simulink model "ElectroMechanics_Q"  (R2024b)
settings: Solver=VariableStepAuto  StartTime=0.0  StopTime=10.0  RelTol=1e-3
libraries: fl_lib x5, nesl_utility x5, sdl_lib x1, batteryecm_lib x1, ee_lib x1
settings Model: Creator=hp  LastModifiedBy=hp

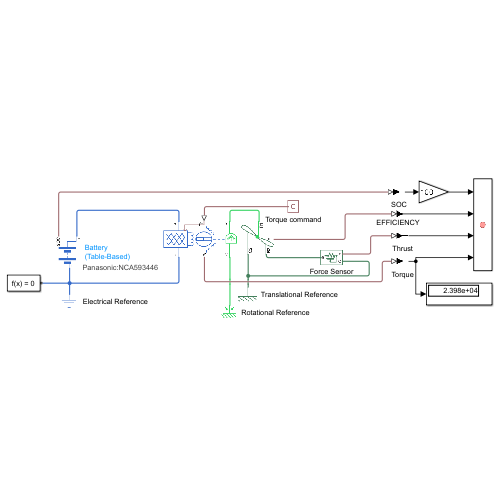
[thumbnail: Simulink's stored preview of the top-level diagram]
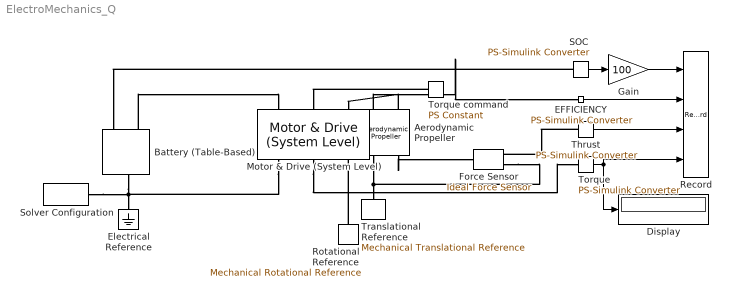
== system ElectroMechanics_Q ==
  " Electrical Reference" : fl_lib/Electrical/Electrical Elements/Electrical Reference
  Aerodynamic Propeller : sdl_lib/Engines & Motors/Aerodynamic Propeller  parameterization=sdl.enum.AerodynamicPropellerParameterization.Constant  pitch_type=foundation.enum.constant_controlled.constant  direction=sdl.enum.PropellerDirection.Positive  root_pitch=0 deg  D=.057 m  kt_const=.1  kp_const=.05  kt_poly_fixed=[.002, .0006, -.0509, .0617]  kp_poly_fixed=[-.0752, .0577, -.0622, .16]  pitch_angle_TLU=[-15, 15, 25, 35, 45] deg  kt_poly_TLU=[.0002, -.00041, -.036, .03; .00026, -.00056, -.048, .04; .002, .00063, -.051, .062; .0014, -.0016, -.048, .087; .00087, -.0036, -.041, .12]  kp_poly_TLU=[-.1, .031, .0055, .088; -.081, -.025, .0044, .07; -.075, .058, -.062, .16; -.052, .065, -.08, .3; -.031, .057, -.069, .4]  J_TLU=[.01, .3, .625, 1.55, 2, 2.6]  kt_TLU_1D=[.0614, .0473, .0318, -.0127, -.0343, -.063]  kp_TLU_1D=[.1496, .1314, .116, -.0521, -.1503, -.2813]  kt_TLU_2D=[.00019, .013, .0048, -.017, -.03, -.045; .00039, .025, .0096, -.037, -.06, -.09; .00061, .047, .032, -.013, -.034, -.063; .00086, .072, .057, .014, -.0076, -.036; .12, .104, .09, .049, .029, .0019]  kp_TLU_2D=[.029, .029, .016, .06, .009, -.16; .059, .054, .031, -.12, -.19, -.29; .15, .13, .12, -.052, -.15, -.28; .26, .24, .22, .097, -.04, -.25; .39, .39, .38, .32, .24, .062]  beta_TLU=linspace(0, 360, 10) deg  Ct_TLU_1D=0.035 * sind(linspace(0, 360, 10) - 200)  Cq_TLU_1D=0.010 * sind(linspace(0, 360, 10) - 200)  Ct_TLU_2D=[0.01 * sind(linspace(0, 360, 10) - 200); 0.020 * sind(linspace(0, 360, 10) - 200); 0.035 * sind(linspace(0, 360, 10) - 200); 0.04 * sind(linspace(0, 360, 10) - 200); 0.06 * sind(linspace(0, 360, 10) - 200)]  Cq_TLU_2D=[0.0005 * sind(linspace(0, 360, 10) - 200); 0.0015 * sind(linspace(0, 360, 10) - 200); 0.0025 * sind(linspace(0, 360, 10) - 200); 0.0035 * sind(linspace(0, 360, 10) - 200); 0.0045 * sind(linspace(0, 360, 10) - 200)]  n_blades=2  n_blade_discretization=20  radial_TLU=[.1, .12, .2, .4, .6, .8, 1]  twist_TLU=[30, 35, 50, 30, 20, 15, 10] deg  chord_TLU=[.0676, .0666, .0824, .1025, .0885, .0598, .0133]  alpha_TLU=-180 : 10 : 180 deg  Cl_TLU=[.1326, .1326, .1274, .1274, .1274, .1274, .1274; .3626, .3626, .5002, .5002, .5002, .5002, .5002; .5528, .5528, .8007, .8007, .8007, .8007, .8007; .7256, .7256, 1.0125, 1.0125, 1.0125, 1.0125, 1.0125; .8016, .8016, 1.1556, 1.1556, 1.1556, 1.1556, 1.1556; .7873, .7873, 1.1604, 1.1604, 1.1604, 1.1604, 1.1604; .7031, .7031, 1.0493, 1.0493, 1.0493, 1.0493, 1.0493; .5423, .5423, .7973, .7973, .7973, .7973, .7973; .3537, .3537, .4332, .4332, .4332, .4332, .4332; .1155, .1155, -.0376, -.0376, -.0376, -.0376, -.0376; -.1045, -.1045, -.4096, -.4096, -.4096, -.4096, -.4096; -.2999, -.2999, -.672, -.672, -.672, -.672, -.672; -.4401, -.4401, -.9343, -.9343, -.9343, -.9343, -.9343; -.5186, -.5186, -1.0477, -1.0477, -1.0477, -1.0477, -1.0477; -.5303, -.5303, -1.0387, -1.0387, -1.0387, -1.0387, -1.0387; -.5073, -.5073, -.9565, -.9565, -.9565, -.9565, -.9565; -.442, -.442, -.7713, -.7713, -.7713, -.7713, -.7713; -.2658, -.2658, -.4832, -.4832, -.4832, -.4832, -.4832; .4109, .4109, .3629, .3629, .3629, .3629, .3629; 1.1635, 1.1635, 1.3779, 1.3779, 1.3779, 1.3779, 1.3779; 1.2412, 1.2412, 1.4033, 1.4033, 1.4033, 1.4033, 1.4033; .7434, .7434, 1.3453, 1.3453, 1.3453, 1.3453, 1.3453; .7908, .7908, 1.2862, 1.2862, 1.2862, 1.2862, 1.2862; .7525, .7525, 1.1562, 1.1562, 1.1562, 1.1562, 1.1562; .6722, .6722, .9487, .9487, .9487, .9487, .9487; .5324, .5324, .7047, .7047, .7047, .7047, .7047; .3365, .3365, .382, .382, .382, .382, .382; .0529, .0529, -.0229, -.0229, -.0229, -.0229, -.0229; -.2728, -.2728, -.316, -.316, -.316, -.316, -.316; -.4135, -.4135, -.6195, -.6195, -.6195, -.6195, -.6195; -.5087, -.5087, -.7847, -.7847, -.7847, -.7847, -.7847; -.5342, -.5342, -.8419, -.8419, -.8419, -.8419, -.8419; -.5166, -.5166, -.7658, -.7658, -.7658, -.7658, -.7658; -.4321, -.4321, -.5707, -.5707, -.5707, -.5707, -.5707; -.2864, -.2864, -.3098, -.3098, -.3098, -.3098, -.3098; -.1073, -.1073, -.0893, -.0893, -.0893, -.0893, -.0893; .1326, .1326, .1274, .1274, .1274, .1274, .1274]  Cd_TLU=[.0055, .0055, .3904, .3904, .3904, .3904, .3904; .0774, .0774, .449, .449, .449, .449, .449; .2412, .2412, .5915, .5915, .5915, .5915, .5915; .4342, .4342, .8307, .8307, .8307, .8307, .8307; .679, .679, 1.0909, 1.0909, 1.0909, 1.0909, 1.0909; .9003, .9003, 1.3868, 1.3868, 1.3868, 1.3868, 1.3868; 1.0825, 1.0825, 1.6565, 1.6565, 1.6565, 1.6565, 1.6565; 1.2281, 1.2281, 1.875, 1.875, 1.875, 1.875, 1.875; 1.3205, 1.3205, 2.017, 2.017, 2.017, 2.017, 2.017; 1.3234, 1.3234, 2.0407, 2.0407, 2.0407, 2.0407, 2.0407; 1.2391, 1.2391, 1.9513, 1.9513, 1.9513, 1.9513, 1.9513; 1.0963, 1.0963, 1.7643, 1.7643, 1.7643, 1.7643, 1.7643; .8978, .8978, 1.5048, 1.5048, 1.5048, 1.5048, 1.5048; .6525, .6525, 1.2281, 1.2281, 1.2281, 1.2281, 1.2281; .4203, .4203, .838, .838, .838, .838, .838; .2428, .2428, .5434, .5434, .5434, .5434, .5434; .0951, .0951, .2517, .2517, .2517, .2517, .2517; .0292, .0292, .0698, .0698, .0698, .0698, .0698; .0148, .0148, .0267, .0267, .0267, .0267, .0267; .0808, .0808, .0509, .0509, .0509, .0509, .0509; .2429, .2429, .1561, .1561, .1561, .1561, .1561; .5019, .5019, .3927, .3927, .3927, .3927, .3927; .7217, .7217, .7438, .7438, .7438, .7438, .7438; .9336, .9336, 1.1277, 1.1277, 1.1277, 1.1277, 1.1277; 1.0984, 1.0984, 1.4838, 1.4838, 1.4838, 1.4838, 1.4838; 1.2274, 1.2274, 1.7877, 1.7877, 1.7877, 1.7877, 1.7877; 1.3016, 1.3016, 1.9779, 1.9779, 1.9779, 1.9779, 1.9779; 1.3305, 1.3305, 2.0516, 2.0516, 2.0516, 2.0516, 2.0516; 1.2889, 1.2889, 1.9974, 1.9974, 1.9974, 1.9974, 1.9974; 1.1677, 1.1677, 1.8463, 1.8463, 1.8463, 1.8463, 1.8463; 1.0076, 1.0076, 1.5699, 1.5699, 1.5699, 1.5699, 1.5699; .8068, .8068, 1.2596, 1.2596, 1.2596, 1.2596, 1.2596; .5688, .5688, .9493, .9493, .9493, .9493, .9493; .3604, .3604, .6154, .6154, .6154, .6154, .6154; .1802, .1802, .5015, .5015, .5015, .5015, .5015; .0699, .0699, .4265, .4265, .4265, .4265, .4265; .0055, .0055, .3904, .3904, .3904, .3904, .3904]  interp_method=simscape.enum.interpolation.linear  extrap_method=simscape.enum.extrapolation.linear  density_spec=foundation.enum.constant_variable.constant  rho=1.225 kg/m^3  rotational_ports=sdl.enum.ConnectionType.Conserving  translational_ports=sdl.enum.ConnectionType.Conserving  model_inertia=true  propeller_inertia=1.5e-7 kg*m^2  propeller_mass=.5 g  efficiency_sensor=true  n_thr=0.001 Hz  k_thr=0.001  P_thr=0.01 W  operation_check=simscape.enum.assert.action.warn  expose_port_C=false  w_specify=off  w_priority=None  w=0 rad/s  w_nominal_specify=off  w_nominal_value=1  w_nominal_unit=rad/s  Q_specify=off  Q_priority=None  Q=0 N*m  Q_nominal_specify=off  Q_nominal_value=1  Q_nominal_unit=N*m  v_specify=off  v_priority=None  v=0 m/s  v_nominal_specify=off  v_nominal_value=1  v_nominal_unit=m/s  thrust_specify=off  thrust_priority=None  thrust=0 N  thrust_nominal_specify=on  thrust_nominal_value=1  thrust_nominal_unit=N
      settings: InternalSimscapePortConfiguration="{\"Bottom\":[],\"Left\":[{\"id\":\"R1\",\"label\":\"R1\",\"type\":\"foundation.mechanical.rotational.rotational\"}],\"Right\":[{\"id\":\"R2\",\"label\":\"R2\",\"type\":\"foundation.mechanical.translational.translational\"},{\"id\":\"C2\",\"label\":\"C2\",\"type\":\"foundation.mechanical.translational.translational\"}],\"Top\":[{\"id\":\"Eff_out\",\"label\":\"E\",\"type\":\"output\"}]}"
  Battery (Table-Based) : batteryecm_lib/Battery (Table-Based)  PartSpecification="{\"DatasetId\":\"Panasonic|NCA593446|simscape.battery.batteryTableBased\",\"DisplayName\":\"Panasonic:NCA593446\"}"  SOC_vec=[0 0.01 0.02 0.03 0.04 0.05 0.06 0.07 0.08 0.09 0.1 0.11 0.12 0.13 0.14 0.15 0.16 0.17 0.18 0.19 0.2 0.21 0.22 0.23 0.24 0.25 0.26 0.27 0.28 0.29 0.3 0.31 0.32 0.33 0.34 0.35 0.36 0.37 0.38 0.39 0.4 0.41 0.42 0.43 0.44 0.45 0.46 0.47 0.48 0.49 0.5 0.51 0.52 0.53 0.54 0.55 0.56 0.57 0.58 0.59 0.6 0.61 0.62 0.63 0.64 0.65 0.66 0.67 0.68 0.69 0.7 0.71 0.72 0.73 0.74 0.75 0.76 0.77 0.78 0.79 0.8 0.81 0.82 0.83 0.84 0.85 0.86 0.87 0.88 0.89 0.9 0.91 0.92 0.93 0.94 0.95 0.96 0.97 0.98 0.99 1] % Datasheet derived  T_dependence=simscape.enum.tablebattery.temperature_dependence.yes  prm_dir=simscape.enum.tablebattery.prm_dir.noCurrentDirectionality  T_vec=[-20 -10 0 25 40] % Datasheet derived degC  V0_mat=[2.84768 2.84768 2.84768 2.84768 2.84768;2.96826 2.96826 2.96826 2.96826 2.96826;3.06574 3.06574 3.06574 3.06574 3.06574;3.13766 3.13766 3.13766 3.13766 3.13766;3.1967 3.1967 3.1967 3.1967 3.1967;3.24166 3.24166 3.24166 3.24166 3.24166;3.27473 3.27473 3.27473 3.27473 3.27473;3.30127 3.30127 3.30127 3.30127 3.30127;3.32686 3.32686 3.32686 3.32686 3.32686;3.34997 3.34997 3.34997 3.34997 3.34997;3.37005 3.37005 3.37005 3.37005 3.37005;3.38547 3.38547 3.38547 3.38547 3.38547;3.39998 3.39998 3.39998 3.39998 3.39998;3.41477 3.41477 3.41477 3.41477 3.41477;3.42833 3.42833 3.42833 3.42833 3.42833;3.4411 3.4411 3.4411 3.4411 3.4411;3.45204 3.45204 3.45204 3.45204 3.45204;3.46216 3.46216 3.46216 3.46216 3.46216;3.47107 3.47107 3.47107 3.47107 3.47107;3.47798 3.47798 3.47798 3.47798 3.47798;3.48476 3.48476 3.48476 3.48476 3.48476;3.49146 3.49146 3.49146 3.49146 3.49146;3.49846 3.49846 3.49846 3.49846 3.49846;3.50538 3.50538 3.50538 3.50538 3.50538;3.51196 3.51196 3.51196 3.51196 3.51196;3.51856 3.51856 3.51856 3.51856 3.51856;3.52563 3.52563 3.52563 3.52563 3.52563;3.53269 3.53269 3.53269 3.53269 3.53269;3.53975 3.53975 3.53975 3.53975 3.53975;3.5468 3.5468 3.5468 3.5468 3.5468;3.55304 3.55304 3.55304 3.55304 3.55304;3.5585 3.5585 3.5585 3.5585 3.5585;3.56345 3.56345 3.56345 3.56345 3.56345;3.56808 3.56808 3.56808 3.56808 3.56808;3.57208 3.57208 3.57208 3.57208 3.57208;3.57682 3.57682 3.57682 3.57682 3.57682;3.58157 3.58157 3.58157 3.58157 3.58157;3.58747 3.58747 3.58747 3.58747 3.58747;3.59339 3.59339 3.59339 3.59339 3.59339;3.59973 3.59973 3.59973 3.59973 3.59973;3.6062 3.6062 3.6062 3.6062 3.6062;3.61263 3.61263 3.61263 3.61263 3.61263;3.61836 3.61836 3.61836 3.61836 3.61836;3.62359 3.62359 3.62359 3.62359 3.62359;3.62865 3.62865 3.62865 3.62865 3.62865;3.63358 3.63358 3.63358 3.63358 3.63358;3.63894 3.63894 3.63894 3.63894 3.63894;3.64566 3.64566 3.64566 3.64566 3.64566;3.65241 3.65241 3.65241 3.65241 3.65241;3.65921 3.65921 3.65921 3.65921 3.65921;3.66761 3.66761 3.66761 3.66761 3.66761;3.67554 3.67554 3.67554 3.67554 3.67554;3.68378 3.68378 3.68378 3.68378 3.68378;3.69229 3.69229 3.69229 3.69229 3.69229;3.70107 3.70107 3.70107 3.70107 3.70107;3.71105 3.71105 3.71105 3.71105 3.71105;3.72105 3.72105 3.72105 3.72105 3.72105;3.73022 3.73022 3.73022 3.73022 3.73022;3.73836 3.73836 3.73836 3.73836 3.73836;3.74563 3.74563 3.74563 3.74563 3.74563;3.75278 3.75278 3.75278 3.75278 3.75278;3.7608 3.7608 3.7608 3.7608 3.7608;3.77031 3.77031 3.77031 3.77031 3.77031;3.78086 3.78086 3.78086 3.78086 3.78086;3.7914 3.7914 3.7914 3.7914 3.7914;3.80194 3.80194 3.80194 3.80194 3.80194;3.81187 3.81187 3.81187 3.81187 3.81187;3.82008 3.82008 3.82008 3.82008 3.82008;3.8281 3.8281 3.8281 3.8281 3.8281;3.83612 3.83612 3.83612 3.83612 3.83612;3.84414 3.84414 3.84414 3.84414 3.84414;3.85216 3.85216 3.85216 3.85216 3.85216;3.86049 3.86049 3.86049 3.86049 3.86049;3.86887 3.86887 3.86887 3.86887 3.86887;3.87725 3.87725 3.87725 3.87725 3.87725;3.88563 3.88563 3.88563 3.88563 3.88563;3.89423 3.89423 3.89423 3.89423 3.89423;3.9041 3.9041 3.9041 3.9041 3.9041;3.91381 3.91381 3.91381 3.91381 3.91381;3.92353 3.92353 3.92353 3.92353 3.92353;3.93322 3.93322 3.93322 3.93322 3.93322;3.94362 3.94362 3.94362 3.94362 3.94362;3.95435 3.95435 3.95435 3.95435 3.95435;3.96525 3.96525 3.96525 3.96525 3.96525;3.97673 3.97673 3.97673 3.97673 3.97673;3.98856 3.98856 3.98856 3.98856 3.98856;4.00085 4.00085 4.00085 4.00085 4.00085;4.01324 4.01324 4.01324 4.01324 4.01324;4.02548 4.02548 4.02548 4.02548 4.02548;4.03638 4.03638 4.03638 4.03638 4.03638;4.04647 4.04647 4.04647 4.04647 4.04647;4.05605 4.05605 4.05605 4.05605 4.05605;4.06452 4.06452 4.06452 4.06452 4.06452;4.07272 4.07272 4.07272 4.07272 4.07272;4.08092 4.08092 4.08092 4.08092 4.08092;4.09076 4.09076 4.09076 4.09076 4.09076;4.1031 4.1031 4.1031 4.1031 4.1031;4.11565 4.11565 4.11565 4.11565 4.11565;4.12892 4.12892 4.12892 4.12892 4.12892;4.15272 4.15272 4.15272 4.15272 4.15272;4.17509 4.17509 4.17509 4.17509 4.17509] % Datasheet derived V  V0_vec=[2.84768 2.96826 3.06574 3.13766 3.1967 3.24166 3.27473 3.30127 3.32686 3.34997 3.37005 3.38547 3.39998 3.41477 3.42833 3.4411 3.45204 3.46216 3.47107 3.47798 3.48476 3.49146 3.49846 3.50538 3.51196 3.51856 3.52563 3.53269 3.53975 3.5468 3.55304 3.5585 3.56345 3.56808 3.57208 3.57682 3.58157 3.58747 3.59339 3.59973 3.6062 3.61263 3.61836 3.62359 3.62865 3.63358 3.63894 3.64566 3.65241 3.65921 3.66761 3.67554 3.68378 3.69229 3.70107 3.71105 3.72105 3.73022 3.73836 3.74563 3.75278 3.7608 3.77031 3.78086 3.7914 3.80194 3.81187 3.82008 3.8281 3.83612 3.84414 3.85216 3.86049 3.86887 3.87725 3.88563 3.89423 3.9041 3.91381 3.92353 3.93322 3.94362 3.95435 3.96525 3.97673 3.98856 4.00085 4.01324 4.02548 4.03638 4.04647 4.05605 4.06452 4.07272 4.08092 4.09076 4.1031 4.11565 4.12892 4.15272 4.17509] % Datasheet derived V  V_range=[2.475 Inf] % Datasheet derived V  R0_mat=[1.17152 1.25921 0.69508 0.13304 0.07171;1.17152 1.25921 1.0047 0.16124 0.03357;1.17152 1.25921 0.97374 0.17824 0.03753;1.17152 1.25921 0.94277 0.18397 0.03713;1.17152 1.25921 0.91181 0.1856 0.05177;1.17152 1.25921 0.88084 0.18421 0.05939;1.17152 1.25921 0.84988 0.17878 0.06959;1.17152 1.25921 0.81891 0.17634 0.07461;1.17152 1.25921 0.78795 0.174 0.0797;1.17152 1.25921 0.75698 0.17214 0.08635;1.17152 1.25921 0.72602 0.17223 0.0906;1.17152 1.25921 0.69505 0.17054 0.09115;1.17152 1.25921 0.66409 0.16925 0.09318;1.17152 1.22525 0.63312 0.16875 0.09628;1.17152 1.19128 0.60216 0.16787 0.0984;1.17152 1.15732 0.57119 0.16678 0.09989;1.17152 1.12335 0.54023 0.16513 0.10147;1.17152 1.08939 0.50867 0.16406 0.10281;1.17152 1.05543 0.47797 0.1625 0.10317;1.17152 1.02146 0.45459 0.15994 0.10196;1.17152 0.9875 0.43292 0.15714 0.10068;1.17152 0.95353 0.41305 0.15431 0.1;1.17152 0.91957 0.39342 0.15202 0.09955;1.17152 0.8856 0.37945 0.15067 0.09904;1.17152 0.85164 0.36632 0.14936 0.09823;1.17152 0.81767 0.35357 0.14805 0.09731;1.17152 0.78371 0.34176 0.14694 0.09677;1.17152 0.74975 0.33164 0.14582 0.09621;1.17152 0.71578 0.32415 0.14471 0.09565;1.17152 0.68182 0.31666 0.1436 0.0951;1.17152 0.64785 0.30853 0.14232 0.09389;1.17152 0.61389 0.3006 0.1409 0.09207;1.17152 0.58003 0.29425 0.13954 0.08984;1.17152 0.55268 0.28763 0.13803 0.08736;1.17152 0.52745 0.28052 0.13616 0.08533;1.17152 0.50643 0.27473 0.13458 0.08451;1.17152 0.48959 0.26905 0.133 0.08369;1.17152 0.47408 0.26428 0.1317 0.0838;1.13618 0.45924 0.26068 0.13039 0.08392;1.10083 0.44473 0.25775 0.12929 0.08436;1.06549 0.43413 0.25494 0.12827 0.0845;1.03015 0.42448 0.25209 0.12722 0.08303;0.99481 0.41337 0.2484 0.12629 0.081;0.95946 0.39916 0.24286 0.12491 0.07858;0.92412 0.38482 0.23717 0.12342 0.07601;0.88878 0.37516 0.23139 0.12187 0.07336;0.85344 0.36733 0.22594 0.12033 0.07168;0.8181 0.3606 0.22242 0.11873 0.07131;0.78275 0.35376 0.21949 0.11718 0.07096;0.74741 0.34688 0.21659 0.11566 0.07065;0.71207 0.34128 0.21496 0.11527 0.07161;0.67646 0.3359 0.21296 0.11494 0.07097;0.6411 0.33115 0.21127 0.11474 0.07051;0.61079 0.32663 0.21087 0.11476 0.07027;0.59072 0.32333 0.21068 0.11496 0.07026;0.5716 0.32098 0.21144 0.11526 0.07193;0.5582 0.31868 0.21222 0.11533 0.07363;0.54553 0.31584 0.20998 0.11502 0.07466;0.53204 0.31219 0.20683 0.11406 0.07488;0.52092 0.30767 0.20299 0.11322 0.07396;0.51011 0.30183 0.19905 0.11239 0.0719;0.49999 0.29668 0.19611 0.11191 0.07053;0.49153 0.29435 0.19583 0.11181 0.07035;0.48648 0.29403 0.19637 0.11212 0.07098;0.48144 0.2937 0.19692 0.11243 0.07169;0.47639 0.29228 0.19768 0.11273 0.07255;0.47086 0.29008 0.19809 0.11274 0.07292;0.46482 0.28706 0.19713 0.11223 0.07194;0.45881 0.28399 0.19601 0.11174 0.0708;0.45281 0.28092 0.19465 0.11125 0.07026;0.4468 0.27841 0.1932 0.11076 0.0702;0.44186 0.27766 0.19175 0.11026 0.07014;0.43883 0.27716 0.19067 0.1097 0.07033;0.43585 0.2767 0.18977 0.109 0.07055;0.43286 0.27697 0.18888 0.10829 0.06994;0.42988 0.27737 0.18801 0.10759 0.06884;0.42716 0.27796 0.18809 0.10696 0.06792;0.42719 0.27952 0.18917 0.10676 0.06801;0.4271 0.28089 0.19026 0.10632 0.06797;0.427 0.28226 0.19163 0.10587 0.06775;0.42689 0.28381 0.19299 0.10543 0.06729;0.42734 0.28617 0.19479 0.10539 0.06739;0.4309 0.28879 0.1967 0.10551 0.06776;0.43574 0.29186 0.19874 0.10565 0.06825;0.44105 0.29582 0.20133 0.10572 0.06922;0.44662 0.30005 0.20423 0.10597 0.06887;0.45424 0.30573 0.20765 0.10644 0.06884;0.46314 0.31211 0.21211 0.10737 0.06889;0.47191 0.31909 0.21644 0.10834 0.06882;0.48274 0.32634 0.22066 0.10863 0.0687;0.49536 0.33329 0.22557 0.10782 0.06813;0.50758 0.34104 0.23008 0.10669 0.06715;0.5236 0.3479 0.23323 0.10518 0.06566;0.54204 0.3557 0.23574 0.1035 0.06457;0.56047 0.36586 0.23825 0.10174 0.06347;0.58089 0.37733 0.24177 0.10038 0.0629;0.60472 0.38891 0.24721 0.10004 0.06261;0.62405 0.40064 0.25192 0.09769 0.06249;0.62609 0.409 0.25687 0.09524 0.05997;0.62318 0.41456 0.2608 0.09028 0.06497;0.61334 0.40006 0.23403 0.07584 0.04513] % Datasheet derived Ohm  R0_vec=[0.13304 0.16124 0.17824 0.18397 0.1856 0.18421 0.17878 0.17634 0.174 0.17214 0.17223 0.17054 0.16925 0.16875 0.16787 0.16678 0.16513 0.16406 0.1625 0.15994 0.15714 0.15431 0.15202 0.15067 0.14936 0.14805 0.14694 0.14582 0.14471 0.1436 0.14232 0.1409 0.13954 0.13803 0.13616 0.13458 0.133 0.1317 0.13039 0.12929 0.12827 0.12722 0.12629 0.12491 0.12342 0.12187 0.12033 0.11873 0.11718 0.11566 0.11527 0.11494 0.11474 0.11476 0.11496 0.11526 0.11533 0.11502 0.11406 0.11322 0.11239 0.11191 0.11181 0.11212 0.11243 0.11273 0.11274 0.11223 0.11174 0.11125 0.11076 0.11026 0.1097 0.109 0.10829 0.10759 0.10696 0.10676 0.10632 0.10587 0.10543 0.10539 0.10551 0.10565 0.10572 0.10597 0.10644 0.10737 0.10834 0.10863 0.10782 0.10669 0.10518 0.1035 0.10174 0.10038 0.10004 0.09769 0.09524 0.09028 0.07584] % Datasheet derived Ohm  R0_dis_mat=[.0117, .0085, .009; .011, .0085, .009; .0114, .0087, .0092; .0107, .0082, .0088; .0107, .0083, .0091; .0113, .0085, .0089; .0116, .0085, .0089] % Parameter not set Ohm  R0_dis_vec=[.0085, .0085, .0087, .0082, .0083, .0085, .0085] % Parameter not set Ohm  R0_ch_mat=[.0117, .0085, .009; .011, .0085, .009; .0114, .0087, .0092; .0107, .0082, .0088; .0107, .0083, .0091; .0113, .0085, .0089; .0116, .0085, .0089] % Parameter not set Ohm  R0_ch_vec=[.0085, .0085, .0087, .0082, .0083, .0085, .0085] % Parameter not set Ohm  AH=1.257 % Datasheet derived hr*A  prm_leak=simscape.enum.tablebattery.prm_leak.disabled  Rleak_vec=[8000, 7000, 6000] % Parameter not set Ohm  Rleak=7e3 % Parameter not set Ohm  extrapolation_option=simscape.enum.extrapolation.nearest  SOC_port=simscape.enum.tablebattery.enable.yes  prm_dyn=simscape.enum.tablebattery.prm_dyn.off  R1_mat=[.0109, .0029, .0013; .0069, .0024, .0012; .0047, .0026, .0013; .0034, .0016, .001; .0033, .0023, .0014; .0033, .0018, .0011; .0028, .0017, .0011] % Parameter not set Ohm  R1_vec=[.0029, .0024, .0026, .0016, .0023, .0018, .0017] % Parameter not set Ohm  tau1_mat=[20, 36, 39; 31, 45, 39; 109, 105, 61; 36, 29, 26; 59, 77, 67; 40, 33, 29; 25, 39, 33] % Parameter not set s  tau1_vec=[36, 45, 105, 29, 77, 33, 39] % Parameter not set s  R2_mat=[.0109, .0029, .0013; .0069, .0024, .0012; .0047, .0026, .0013; .0034, .0016, .001; .0033, .0023, .0014; .0033, .0018, .0011; .0028, .0017, .0011] % Parameter not set Ohm  R2_vec=[.0029, .0024, .0026, .0016, .0023, .0018, .0017] % Parameter not set Ohm  tau2_mat=[20, 36, 39; 31, 45, 39; 109, 105, 61; 36, 29, 26; 59, 77, 67; 40, 33, 29; 25, 39, 33] % Parameter not set s  tau2_vec=[36, 45, 105, 29, 77, 33, 39] % Parameter not set s  R3_mat=[.0109, .0029, .0013; .0069, .0024, .0012; .0047, .0026, .0013; .0034, .0016, .001; .0033, .0023, .0014; .0033, .0018, .0011; .0028, .0017, .0011] % Parameter not set Ohm  R3_vec=[.0029, .0024, .0026, .0016, .0023, .0018, .0017] % Parameter not set Ohm  tau3_mat=[20, 36, 39; 31, 45, 39; 109, 105, 61; 36, 29, 26; 59, 77, 67; 40, 33, 29; 25, 39, 33] % Parameter not set s  tau3_vec=[36, 45, 105, 29, 77, 33, 39] % Parameter not set s  R4_mat=[.0109, .0029, .0013; .0069, .0024, .0012; .0047, .0026, .0013; .0034, .0016, .001; .0033, .0023, .0014; .0033, .0018, .0011; .0028, .0017, .0011] % Parameter not set Ohm  R4_vec=[.0029, .0024, .0026, .0016, .0023, .0018, .0017] % Parameter not set Ohm  tau4_mat=[20, 36, 39; 31, 45, 39; 109, 105, 61; 36, 29, 26; 59, 77, 67; 40, 33, 29; 25, 39, 33] % Parameter not set s  tau4_vec=[36, 45, 105, 29, 77, 33, 39] % Parameter not set s  R5_mat=[.0109, .0029, .0013; .0069, .0024, .0012; .0047, .0026, .0013; .0034, .0016, .001; .0033, .0023, .0014; .0033, .0018, .0011; .0028, .0017, .0011] % Parameter not set Ohm  R5_vec=[.0029, .0024, .0026, .0016, .0023, .0018, .0017] % Parameter not set Ohm  tau5_mat=[20, 36, 39; 31, 45, 39; 109, 105, 61; 36, 29, 26; 59, 77, 67; 40, 33, 29; 25, 39, 33] % Parameter not set s  tau5_vec=[36, 45, 105, 29, 77, 33, 39] % Parameter not set s  prm_fade=simscape.enum.tablebattery.prm_fade.tableN  N0=100 % Parameter not set  dV0=0 % Parameter not set  dR0=0 % Parameter not set  dAH=0 % Parameter not set  dRleak=0 % Parameter not set  dR1=0 % Parameter not set  dR2=0 % Parameter not set  dR3=0 % Parameter not set  dR4=0 % Parameter not set  dR5=0 % Parameter not set  N0vec=[0 6 11 16 21 26 31 36 41 46 51 56 61 66 71 76 81 86 91 96 101 106 111 116 121 126 131 136 141 146 151 156 161 166 171 176 181 186 191 196 201 206 211 216 221 226 231 236 241 246 251 256 261 266 271 276 281 286 291 296 301 306 311 316 321 326 331 336 341 346 351 356 361 366 371 376 381 386 391 396 401 406 411 416 421 426 431 436 441 446 451 456 461 466 471 476 481 486 491] % Datasheet derived  Tfadevec=[298.15, 323.15] % Parameter not set K  dV0vec=[0 -0.352 -0.7148 -1.0894 -1.2653 -1.3543 -1.4422 -1.5264 -1.6106 -1.6948 -1.778 -1.8424 -1.8912 -1.94 -1.9888 -2.034 -2.0729 -2.1118 -2.1507 -2.1912 -2.2318 -2.2695 -2.3033 -2.3371 -2.3709 -2.405 -2.4395 -2.4741 -2.5088 -2.5434 -2.578 -2.6126 -2.6472 -2.6829 -2.7123 -2.7403 -2.7682 -2.7962 -2.8241 -2.8522 -2.8792 -2.9007 -2.9222 -2.9437 -2.9652 -2.9867 -3.0082 -3.0297 -3.0678 -3.1207 -3.1743 -3.2279 -3.2815 -3.3361 -3.394 -3.4519 -3.4926 -3.5213 -3.5501 -3.5788 -3.6104 -3.6427 -3.6749 -3.7071 -3.7474 -3.7913 -3.8351 -3.879 -3.9235 -3.9624 -3.9985 -4.0347 -4.0709 -4.1071 -4.1433 -4.1828 -4.225 -4.2671 -4.3093 -4.3515 -4.3918 -4.4279 -4.464 -4.4989 -4.5337 -4.5685 -4.6032 -4.638 -4.6711 -4.697 -4.7229 -4.7488 -4.774 -4.7992 -4.8391 -4.8828 -4.9264 -4.97 -5.0136] % Datasheet derived  dR0vec=[0 0 0 0 0 0 0 0 0 0 0 0 0 0 0 0 0 0 0 0 0 0 0 0 0 0 0 0 0 0 0 0 0 0 0 0 0 0 0 0 0 0 0 0 0 0 0 0 0 0 0 0 0 0 0 0 0 0 0 0 0 0 0 0 0 0 0 0 0 0 0 0 0 0 0 0 0 0 0 0 0 0 0 0 0 0 0 0 0 0 0 0 0 0 0 0 0 0 0] % Parameter assumed  dAHvec=[0 -0.657 -1.314 -1.971 -2.502 -2.782 -3.062 -3.342 -3.621 -3.901 -4.181 -4.399 -4.564 -4.729 -4.894 -5.059 -5.225 -5.39 -5.555 -5.727 -5.899 -6.071 -6.243 -6.415 -6.587 -6.761 -6.937 -7.113 -7.289 -7.466 -7.642 -7.818 -7.994 -8.17 -8.316 -8.453 -8.591 -8.729 -8.867 -9.005 -9.122 -9.216 -9.31 -9.403 -9.497 -9.591 -9.684 -9.778 -9.944 -10.165 -10.387 -10.609 -10.831 -11.053 -11.274 -11.496 -11.652 -11.762 -11.872 -11.982 -12.092 -12.202 -12.312 -12.422 -12.559 -12.709 -12.859 -13.008 -13.158 -13.289 -13.411 -13.533 -13.655 -13.777 -13.899 -14.032 -14.176 -14.319 -14.462 -14.605 -14.742 -14.865 -14.988 -15.11 -15.233 -15.356 -15.478 -15.601 -15.718 -15.809 -15.901 -15.992 -16.084 -16.175 -16.32 -16.479 -16.637 -16.796 -16.955] % Datasheet derived  dRleakvec=[0, 0, 0, 0] % Parameter not set  dR1vec=[0, 0, 0, 0] % Parameter not set  dR2vec=[0, 0, 0, 0] % Parameter not set  dR3vec=[0, 0, 0, 0] % Parameter not set  dR4vec=[0, 0, 0, 0] % Parameter not set  dR5vec=[0, 0, 0, 0] % Parameter not set  dV0mat=[0, 0; 0, 0; 0, 0; 0, 0] % Parameter not set  dR0mat=[0, 0; 0, 0; 0, 0; 0, 0] % Parameter not set  dAHmat=[0, 0; 0, 0; 0, 0; 0, 0] % Parameter not set  dRleakmat=[0, 0; 0, 0; 0, 0; 0, 0] % Parameter not set  dR1mat=[0, 0; 0, 0; 0, 0; 0, 0] % Parameter not set  dR2mat=[0, 0; 0, 0; 0, 0; 0, 0] % Parameter not set  dR3mat=[0, 0; 0, 0; 0, 0; 0, 0] % Parameter not set  dR4mat=[0, 0; 0, 0; 0, 0; 0, 0] % Parameter not set  dR5mat=[0, 0; 0, 0; 0, 0; 0, 0] % Parameter not set  prm_age_modeling=simscape.enum.tablebattery.prm_age_modeling.equation  storage_dt_age_vec=[0] % Parameter not set d  storage_T_age_vec=[273] % Parameter not set K  prm_age_OCV=simscape.enum.tablebattery.prm_age_OCV.OCV  OCV_age=0.9 % Parameter not set  SOC_age=0.6 % Parameter not set  prm_age_resistance=simscape.enum.tablebattery.prm_age.disabled  OCV_scaling_age_resistance=2.2134e6 % Parameter not set  OCV_offset_age_resistance=1.632e6 % Parameter not set  temp_exp_age_resistance=0.515833569 % Parameter not set V  t_exp_age_resistance=0.75 % Parameter not set  T_age_vec_resistance=[273.15, 298.15, 323.15] % Parameter not set K  dt_age_vec_resistance=[0, 90, 180, 270] % Parameter not set d  dR0_age_vec=[0, 0, 0] % Parameter not set  t_meas_dR0_age=100 % Parameter not set d  dR0_age_mat=[0, 0, 0; 0, 0, 0; 0, 0, 0; 0, 0, 0] % Parameter not set  prm_age_capacity=simscape.enum.tablebattery.prm_age.disabled  OCV_scaling_age_capacity=1.5097e07 % Parameter not set  OCV_offset_age_capacity=8.3625e06 % Parameter not set  temp_exp_age_capacity=0.6011 % Parameter not set V  t_exp_age_capacity=0.75 % Parameter not set  T_age_vec_capacity=[273.15, 298.15, 323.15] % Parameter not set K  dt_age_vec_capacity=[0, 90, 180, 270] % Parameter not set d  dAH_age_vec=[0, 0, 0] % Parameter not set  t_meas_dAH_age=100 % Parameter not set d  dAH_age_mat=[0, 0, 0; 0, 0, 0; 0, 0, 0; 0, 0, 0] % Parameter not set  thermal_port=simscape.enum.thermaleffects.omit  temperature=298.15 % Parameter not set K  thermal_mass=18.54 % Parameter assumed J/K  i_specify=off  i_priority=None  i=0 A  i_nominal_specify=off  i_nominal_value=1  i_nominal_unit=A  v_specify=off  v_priority=None  v=0 V  v_nominal_specify=off  v_nominal_value=1  v_nominal_unit=V  stateOfCharge_specify=off  stateOfCharge_priority=High  stateOfCharge=1  stateOfCharge_nominal_specify=off  stateOfCharge_nominal_value=1  stateOfCharge_nominal_unit=1  num_cycles_specify=off  num_cycles_priority=High  num_cycles=0  num_cycles_nominal_specify=off  num_cycles_nominal_value=1  num_cycles_nominal_unit=1  cell_temperature_specify=off  cell_temperature_priority=High  cell_temperature=298.15 K  cell_temperature_nominal_specify=off  cell_temperature_nominal_value=1  cell_temperature_nominal_unit=K
      settings: AttributesFormatString=Panasonic:NCA593446  InternalSimscapePortConfiguration="{\"Bottom\":[],\"Left\":[{\"id\":\"p\",\"label\":\"+\",\"type\":\"foundation.electrical.electrical\"},{\"id\":\"soc\",\"label\":\"SOC\",\"type\":\"output\"}],\"Right\":[{\"id\":\"n\",\"label\":\"-\",\"type\":\"foundation.electrical.electrical\"}],\"Top\":[]}"
  Display : Display
  "EFFICIENCY " : nesl_utility/PS-Simulink Converter  PhysicalDomain=network_engine_domain  SubClassName=ps_output  LeftPortType=input  RightPortType=output  PseudoPeriodic=off  Frequencies=[]  VectorFormat=inherit  Unit=V  AffineConversion=off
  Force Sensor : fl_lib/Mechanical/Mechanical Sensors/Ideal Force Sensor
  Gain : Gain  Gain=100
  Motor & Drive (System Level) : ee_lib/Electromechanical/Motor & Drive (System Level)  torque_speed_param=ee.enum.electromech.envelope.torque_power  overtorque_param=ee.enum.electromech.overtorque.no  T_t=[.09, .08, .07, 0] N*m  T_t_intermittent=[.36, .32, .28, 0] N*m  T_t_2D=[.09, .09, .09; .08, .08, .08; .07, .07, .07; 0, 0, 0] N*m  T_t_intermittent_2D=[.36, .36, .36; .32, .32, .32; .28, .28, .28; 0, 0, 0] N*m  w_t=[0, 3750, 7500, 8000] rpm  vdc_t=[6, 12, 24] V  torque_max=1 mN*m  power_max=3 W  torque_max_intermittent=0.4 N*m  power_max_intermittent=120 W  time_overtorque=30 s  time_recover=60 s  Tc=0.02 s  EnableSwitch=false  losses_param=1  eff=74  w_eff=3e4 rpm  T_eff=1 mN*m  Piron=0 W  Pbase=0 W  w_eff_vec=[-8000, -4000, 0, 4000, 8000] rpm  T_eff_vec=[0, .03, .06, .09] N*m  v_eff_vec=[100, 250, 400] V  losses_mat=[1.49, 1.67, 2.21, 3.1; .42, .69, 1.14, 2.03; .06, .24, .78, 1.68; .42, .69, 1.14, 2.03; 1.49, 1.67, 2.21, 3.1] W  efficiency_mat=[95, 95, 95, 95; 95, 95, 95, 95; 95, 95, 95, 95; 95, 95, 95, 95; 95, 95, 95, 95]  losses_mat_3D=ones(5, 4, 3) W  efficiency_mat_3D=95 * ones(5, 4, 3)  Res=0 Ohm  J=8e-9 kg*m^2  lam=2.5e-8 N*m*s/rad  speed0=0 rpm  fault_condition=1  fault_threshold=0.5  faulted_specify=off  faulted_priority=None  faulted=0  faulted_nominal_specify=off  faulted_nominal_value=1  faulted_nominal_unit=1  isSwitchedOff_specify=off  isSwitchedOff_priority=None  isSwitchedOff=0  isSwitchedOff_nominal_specify=off  isSwitchedOff_nominal_value=1  isSwitchedOff_nominal_unit=1  torqueLimitContinuous_specify=off  torqueLimitContinuous_priority=None  torqueLimitContinuous=0 N*m  torqueLimitContinuous_nominal_specify=off  torqueLimitContinuous_nominal_value=1  torqueLimitContinuous_nominal_unit=N*m  alpha=3.93e-3 1/K  Tmeas=25 degC  Tmeas2=125 degC  losses_mat_T2=[1.49, 1.74, 2.49, 3.74; .42, .67, 1.42, 2.67; .06, .31, 1.06, 2.31; .42, .67, 1.42, 2.67; 1.49, 1.74, 2.49, 3.74] W  efficiency_mat_T2=[95, 95, 95, 95; 95, 95, 95, 95; 95, 95, 95, 95; 95, 95, 95, 95; 95, 95, 95, 95]  losses_mat_3D_T2=ones(5, 4, 3) W  efficiency_mat_3D_T2=95 * ones(5, 4, 3)  thermal_mass=100 J/K  initial_temperature=25 degC
  Record : Record  FileSettingsInternal="{\"entries\":[{\"content\":{\"excelSettings\":{\"content\":{},\"type\":\"Streamout.ExcelSettings\"}},\"type\":\"Streamout.FileSettingStorage\",\"uuid\":\"\"}],\"packageUris\":[\"http:\\/\\/schema.mathworks.com\\/mf0\\/streamout_blocks\\/R2020a\"],\"version\":\"1.0\"}"  SignalsInternal="{\"entries\":[{\"content\":{\"signals\":[{\"content\":{\"blockPath\":[],\"dimensions\":[1],\"domain\":\"\",\"lineColor\":\"#7e2f8e\",\"lineStyle\":\"DASH_DOT\",\"lineWidth\":6,\"plots\":[ 1 ],\"port\":1,\"sid\":[\"\"],\"signalID\":1,\"signalName\":\"Gain\"},\"type\":\"RecordBlkView.Signal\",\"uuid\":\"\"},{\"content\":{\"blockPath\":[],\"dimensions\":[1],\"domain\":\"\",\"lineColor\":\"#edb120\",\"lineWidth\":5,\"plots\":[ 1 ],\"port\":2,\"sid\":[\"\"],\"signalID\":2,\"signalName\":\"EFFICIENCY \"},\"type\":\"RecordBlkView.Signal\",\"uuid\":\"\"},{\"content\":{\"blockPath\":[],\"dimensions\":[1],\"domain\":\"\",\"lineColor\":\"#139fff\",\"lineWidth\":2,\"plots\":[ 1 ],\"port\":3,\"sid\":[\"\"],\"signalID\":3,\"signalName\":\"Thrust\"},\"type\":\"RecordBlkView.Signal\",\"uuid\":\"\"},{\"content\":{\"blockPath\":[],\"dimensions\":[1],\"domain\":\"\",\"lineColor\":\"#ff6929\",\"lineWidth\":2,\"plots\":[ 1 ],\"port\":4,\"sid\":[\"\"],\"signalID\":4,\"signalName\":\"Torque\"},\"type\":\"RecordBlkView.Signal\",\"uuid\":\"\"}]},\"type\":\"RecordBlkView.InputSignals\",\"uuid\":\"\"}],\"packageUris\":[\"http:\\/\\/schema.mathworks.com\\/mf0\\/streamout_blocks\\/R2020a\"],\"version\":\"1.0\"}"  VisualizationBindings="{\"sparklinesplugin\":{\"info\":[{\"bindingParametersList\":[],\"subplotID\":1}]}}"
  Rotational Reference : fl_lib/Mechanical/Rotational Elements/Mechanical Rotational Reference
  SOC : nesl_utility/PS-Simulink Converter  PhysicalDomain=network_engine_domain  SubClassName=ps_output  LeftPortType=input  RightPortType=output  PseudoPeriodic=off  Frequencies=[]  VectorFormat=inherit  Unit=inherit  AffineConversion=off
  Solver Configuration : nesl_utility/Solver Configuration  PhysicalDomain=network_engine_domain  SubClassName=solver  LeftPortType=input  RightPortType=generic  Tones=[]  Harmonics=[]  SimulateNoise=off  Profile=off  UseLocalSampling=off  EnableSwitchedLinearOptims=on  FrequencyDomain=off  UseCCode=off  RelTol=0.001  AbsTol=0.001  MinStep=1e-09  ToWorkspace=off  RevertToSquareIcSolve=off  NumHomotopyIterations=100  PhasorMode=off  PhasorModeNumHarmonics=1  ConsistencySolver=NEWTON_XTOL_AFTER_FTOL  IndexReductionMethod=DerivativeReplacement  DoDC=off  ResidualTolerance=1e-09  ConsistencyTolSource=GLOBAL  ConsistencyAbsTol=0.001  ConsistencyRelTol=0.001  ConsistencyTolFactor=0.001  UseLocalSolver=off  LocalSolverChoice=NE_BACKWARD_EULER_ADVANCER  ResolveIndetEquations=on  FunctionEvalNumThread=1  LocalSolverSampleTime=0.001  DoFixedCost=off  MaxNonlinIter=3  MaxModeIter=2  ComputeImpulses=off  ImpulseIterations=2  LinearAlgebra=auto  LinearAlgebraNumThread=0  EquationFormulation=NE_TIME_EF  DelaysMemoryBudget=1024  AutomaticFiltering=on  FilteringTimeConstant=0.001  PartitionStorageMethod=AS_NEEDED  PartitionMemoryBudget=1024  PartitionMethod=ROBUST  MultibodyUseLocalSolver=off  MultibodyLocalSolverChoice=ODE1  MultibodyLocalSolverSampleTime=0.001
  Thrust : nesl_utility/PS-Simulink Converter  PhysicalDomain=network_engine_domain  SubClassName=ps_output  LeftPortType=input  RightPortType=output  PseudoPeriodic=off  Frequencies=[]  VectorFormat=inherit  Unit=inherit  AffineConversion=off
  Torque : nesl_utility/PS-Simulink Converter  PhysicalDomain=network_engine_domain  SubClassName=ps_output  LeftPortType=input  RightPortType=output  PseudoPeriodic=off  Frequencies=[]  VectorFormat=inherit  Unit=rpm  AffineConversion=off
  Torque command : fl_lib/Physical Signals/Sources/PS Constant  constant=1 mN*m
  Translational Reference : fl_lib/Mechanical/Translational Elements/Mechanical Translational Reference
  wires:
  Thrust/1 -> Record/3
  "EFFICIENCY "/1 -> Record/2
  Gain/1 -> Record/1
  Torque/1 -> Display/1, Record/4
  SOC/1 -> Gain/1
  connections:
  Battery (Table-Based)/RConn1 -- Motor & Drive (System Level)/RConn1 -- Solver Configuration/RConn1 -- " Electrical Reference"/LConn1
  Aerodynamic Propeller/LConn1 -- Motor & Drive (System Level)/LConn3
  Aerodynamic Propeller/RConn2 -- Force Sensor/RConn1 -- Translational Reference/LConn1
  Rotational Reference/LConn1 -- Motor & Drive (System Level)/RConn3
  Torque command/RConn1 -- Motor & Drive (System Level)/LConn2
  Battery (Table-Based)/LConn1 -- Motor & Drive (System Level)/LConn1
  Aerodynamic Propeller/RConn1 -- Force Sensor/LConn1
  Thrust/LConn1 -- Force Sensor/RConn2
  Aerodynamic Propeller/LConn2 -- "EFFICIENCY "/LConn1
  Motor & Drive (System Level)/RConn2 -- Torque/LConn1
  SOC/LConn1 -- Battery (Table-Based)/LConn2
